simulink model "sensored_foc_model"  (R2022b)
settings: Solver=ode4  StartTime=0.0  StopTime=1800  FixedStep=50e-6  RelTol=1e-3  EnableMultiTasking=on
undefined symbols (not defined in the file or in its folder): DiscIntNeverNeededParam
libraries: slpidlib x2, spsCurrentMeasurementLib x2, mcbcontrolslib x1, spsDCVoltageSourceLib x1, eePwmGeneratorTwoLevel x1, spsPermanentMagnetSynchronousMachineLib x1, simulink x1, spsUniversalBridgeLib x1, sps_lib x1
settings Model: Creator=ASUS  LastModifiedBy=ASUS
settings SolverCC: PositivePriorityOrder=on
settings OptimizationCC: DefaultParameterBehavior=Inlined  EnhancedBackFolding=on  PassReuseOutputArgsAs=Individual arguments  ZeroExternalMemoryAtStartup=off  ZeroInternalMemoryAtStartup=off  MaxStackSize=64  OptimizeBlockOrder=speed  DifferentSizesBufferReuse=on  OptimizationCustomize=off  EfficientTunableParamExpr=on
settings DebuggingCC: ParameterTunabilityLossMsg=error
settings HardwareCC: ProdBitPerPointer=32  ProdBitPerSizeT=32  ProdBitPerPtrDiffT=32  ProdLargestAtomicFloat=None  ProdWordSize=32  ProdHWDeviceType=Custom Processor->Custom  HardwareBoardFeatureSet=SoCBlockset
settings ModelReferenceCC: ModelReferenceNumInstancesAllowed=Single
settings SFSimCC: MATLABDynamicMemAlloc=off
settings RTWCC: Description=Embedded Coder  SystemTargetFile=ert.tlc  TemplateMakefile=ert_default_tmf  GenerateReport=on  LaunchReport=on
settings CodeAppCC: ForceParamTrailComments=on  IgnoreCustomStorageClasses=off  OperatorAnnotations=on  SimulinkDataObjDesc=on  SFDataObjDesc=on  InsertBlockDesc=on
settings ERTTargetCC: InlinedParameterPlacement=NonHierarchical  ERTCustomFileTemplate=example_file_process.tlc

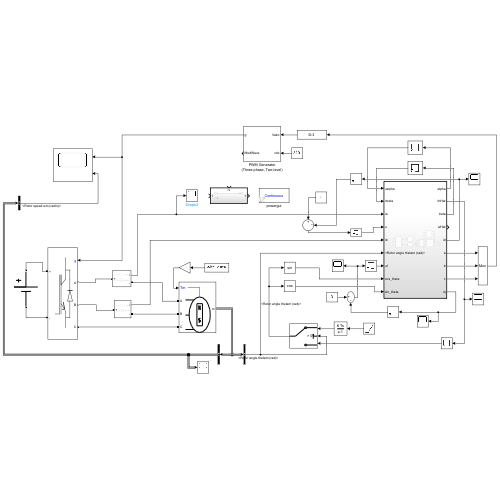
[thumbnail: Simulink's stored preview of the top-level diagram]
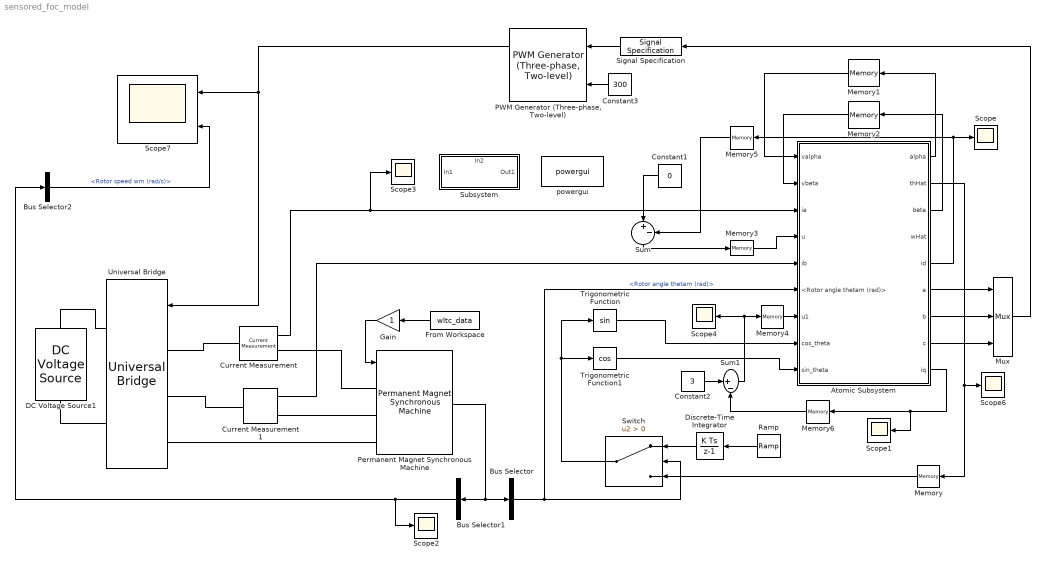
== system sensored_foc_model ==
  Atomic Subsystem : Subsystem  TreatAsAtomicUnit=on
  Bus Selector : BusSelector  OutputSignals=Rotor angle thetam (rad)  OutputAsBus=on
  Bus Selector1 : BusSelector  OutputSignals=Rotor angle thetam (rad),Rotor speed wm (rad/s),Electromagnetic torque Te (N*m)  OutputAsBus=on
  Bus Selector2 : BusSelector  OutputSignals=Rotor speed wm (rad/s)
  Constant1 : Constant  Value=0
  Constant2 : Constant  Value=3
  Constant3 : Constant  Value=300
  Current Measurement : spsCurrentMeasurementLib/Current Measurement  PhasorSimulation=off  OutputType=Complex  PSBequivalent=0
  Current Measurement1 : spsCurrentMeasurementLib/Current Measurement  PhasorSimulation=off  OutputType=Complex  PSBequivalent=0
  DC Voltage Source1 : spsDCVoltageSourceLib/DC Voltage Source  Amplitude=400  Measurements=None
  Discrete-Time Integrator : DiscreteIntegrator  SampleTime=-1  ICPrevOutput=DiscIntNeverNeededParam  ICPrevScaledInput=DiscIntNeverNeededParam
  From Workspace : FromWorkspace  VariableName=wltc_data
  Gain : Gain
  Memory{,1..6} (7 alike) : Memory
  Mux : Mux  Inputs=3
  "PWM Generator (Three-phase, Two-level)" : eePwmGeneratorTwoLevel/PWM Generator (Three-phase, Two-level)  PWMMode=Continuous PWM (CPWM)  CPWMMode=SPWM: sinusoidal PWM  DPWMMode=60 DPWM: 60 degree discontinuous PWM  fsw=1e3  Ts=5e-5
      settings: LibrarySourceBlock=|
      | ee_sl_lib/Pulse Width
      | Modulation/PWM Generator
      | (Three-phase, Two-level)
  Permanent Magnet Synchronous Machine : spsPermanentMagnetSynchronousMachineLib/Permanent Magnet Synchronous Machine  NbPhases=3  FluxDistribution=Sinusoidal  RotorType=Round  MechanicalLoad=Torque Tm  PresetModel=No  ShowDetailedParameters=on  MeasurementBus=off  Resistance=0.0485  Inductance=8.5e-3  dqInductances=[8.5e-3,8.5e-3]  La=0.000395  MachineConstant=Flux linkage established by magnets (V.s)  Flux=0.1194  VoltageCst=86.6271  TorqueCst=0.7164  Flat=120  Mechanical=[0.0027 0.0004924 4 0]  PolePairs=4  InitialConditions=[0,0, 0,0]  InitialConditions5ph=[0 0 0 0 0 0]  RefAngle=90 degrees behind phase A axis (modified Park)  IterativeDiscreteModel=Trapezoidal non iterative  TsBlock=-1  TsPowergui=0
  Ramp : simulink/Sources/Ramp  slope=0.2  start=0  InitialOutput=0
  Scope{,1..4,6} (6 alike) : Scope
  Scope7 : Scope  NumInputPorts=2
  Signal Specification : SignalSpecification  Dimensions=3
  Subsystem : Subsystem  TreatAsAtomicUnit=on
      settings: PortSchema="{\"entries\":[{\"content\":{\"sides\":[{\"content\":{\"connectorIds\":[\"In1\"]},\"type\":\"ConnectorPlacement.EquallySpacedRectSide\",\"uuid\":\"b96b767d-adbf-48c0-96dd-5b9b5a7e8c99\"},{\"content\":{\"connectorIds\":[\"Out1\"],\"side\":\"RIGHT\"},\"type\":\"ConnectorPlacement.EquallySpacedRectSide\",\"uuid\":\"f8319ca3-800b-423a-9674-6b1ed0ebf810\"},{\"content\":{\"connectorIds\":[\"In2\"],\"side\":\"TOP\"},\"type\":\"ConnectorPlacement.EquallySpacedRectSide\",\"uuid\":\"813efe85-bf04-45d5-92e6-bee0d44ebe10\"}]},\"type\":\"ConnectorPlacement.EquallySpacedConnector\",\"uuid\":\"16ba6ebc-7a04-4ed7-9949-8c258e0a29ab\"}],\"packageUris\":[\"http://schema.mathworks.com/mf0/Connector/R2020b\"],\"version\":\"1.0\"}"
      settings: LibrarySourceBlock=|
      | hdlsllib/Ports &
      | Subsystems/Subsystem
  Sum : Sum  Inputs=|+-
  Sum1 : Sum  Inputs=|+-
  Switch : Switch  Criteria=u2 > Threshold  SaturateOnIntegerOverflow=off  InputSameDT=off
  Trigonometric Function : Trigonometry
  Trigonometric Function1 : Trigonometry  Operator=cos
  Universal Bridge : spsUniversalBridgeLib/Universal Bridge  Arms=3  SnubberResistance=1e5  SnubberCapacitance=0  Device=IGBT / Diodes  Ron=1e-3  Lon=0  ForwardVoltages="[  0  0  ]"  ForwardVoltage=0  GTOparameters=[ 10e-6 , 20e-6 ]  IGBTparameters=[ 1e-6 , 2e-6 ]  Measurements=None  Measurements_2=None  converterType=Rectifier
  powergui : sps_lib/powergui  Priority=1  SimulationMode=Continuous  SampleTime=50e-6  frequency=60  Iterations=50  frequencyindice=0  Pbase=100e6  ErrMax=1e-4  UnitsV=kV  UnitsW=MW  buscounter=0  FunctionMessages=off  echomessages=off  EnableUseOfTLC=off  CurrentSourceSwitches=off  DisableSnubberDevices=off  DisableRonSwitches=off  DisableVfSwitches=off  DisplayEquations=off  AutomaticDiscreteSolvers=off  SolverType=Tustin/Backward Euler (TBE)  Interpol=off  ExternalGateDelay=off  methode=off  Ts=100  x0status=blocks  SPID=on  SwTol=0  HookPort=off  NonlinearTolerance=1e-4  nMaxIteration=100  ContinueOnMaxIteration=off  RestoreLinks=warning  ResistiveCurrentMeasurement=off  Frange=[0:2:500]  Ylog=off  Xlog=on  ShowGrid=off  save=off  variable=ZData  structure=0  ZoomFFT=off  StartTime=0.0  cycles=1  DisplayStyle=1  fundamental=60  FreqAxis=off  MaxFrequency=1000  frequencyindicesteady=1  RmsSteady=1  display=off
  wires:
  Atomic Subsystem/6(a) -> Mux/1
  "PWM Generator (Three-phase, Two-level)"/1 -> Scope7/1, Universal Bridge/1
  Signal Specification/1 -> "PWM Generator (Three-phase, Two-level)"/1
  Atomic Subsystem/3(beta) -> Memory2/1
  Mux/1 -> Signal Specification/1
  Current Measurement1/1 -> Atomic Subsystem/5(ib)
  Constant3/1 -> "PWM Generator (Three-phase, Two-level)"/2
  Atomic Subsystem/7(b) -> Mux/2
  Bus Selector/1 -> Switch/2, Atomic Subsystem/6(<Rotor angle thetam (rad)>)  "<Rotor angle thetam (rad)>"
  Trigonometric Function1/1 -> Atomic Subsystem/9(sin_theta)
  Current Measurement/1 -> Scope3/1, Atomic Subsystem/3(ia)
  Ramp/1 -> Discrete-Time Integrator/1
  Atomic Subsystem/8(c) -> Mux/3
  Memory1/1 -> Atomic Subsystem/1(valpha)
  Permanent Magnet Synchronous Machine/1 -> Bus Selector1/1, Bus Selector/1
  Discrete-Time Integrator/1 -> Switch/1
  Switch/1 -> Trigonometric Function/1, Trigonometric Function1/1
  Constant1/1 -> Sum/1
  Memory2/1 -> Atomic Subsystem/2(vbeta)
  Memory/1 -> Switch/3
  Atomic Subsystem/1(alpha) -> Memory1/1
  Atomic Subsystem/9(iq) -> Scope1/1, Memory6/1
  Trigonometric Function/1 -> Atomic Subsystem/8(cos_theta)
  Constant2/1 -> Sum1/1
  Atomic Subsystem/2(thHat) -> Memory/1, Scope6/1
  Atomic Subsystem/5(id) -> Scope/1, Memory5/1
  Memory3/1 -> Atomic Subsystem/4(u)
  Sum/1 -> Memory3/1
  Memory4/1 -> Atomic Subsystem/7(u1)
  Sum1/1 -> Memory4/1, Scope4/1
  Memory5/1 -> Sum/2
  Memory6/1 -> Sum1/2
  Bus Selector1/1 -> Bus Selector2/1, Scope2/1
  Bus Selector2/1 -> Scope7/2  "<Rotor speed wm (rad/s)>"
  From Workspace/1 -> Gain/1
  Gain/1 -> Permanent Magnet Synchronous Machine/1
  connections:
  DC Voltage Source1/LConn1 -- Universal Bridge/RConn2
  DC Voltage Source1/RConn1 -- Universal Bridge/RConn1
  Universal Bridge/LConn1 -- Current Measurement/LConn1
  Universal Bridge/LConn2 -- Current Measurement1/LConn1
  Universal Bridge/LConn3 -- Permanent Magnet Synchronous Machine/LConn3
  Current Measurement/RConn1 -- Permanent Magnet Synchronous Machine/LConn1
  Current Measurement1/RConn1 -- Permanent Magnet Synchronous Machine/LConn2

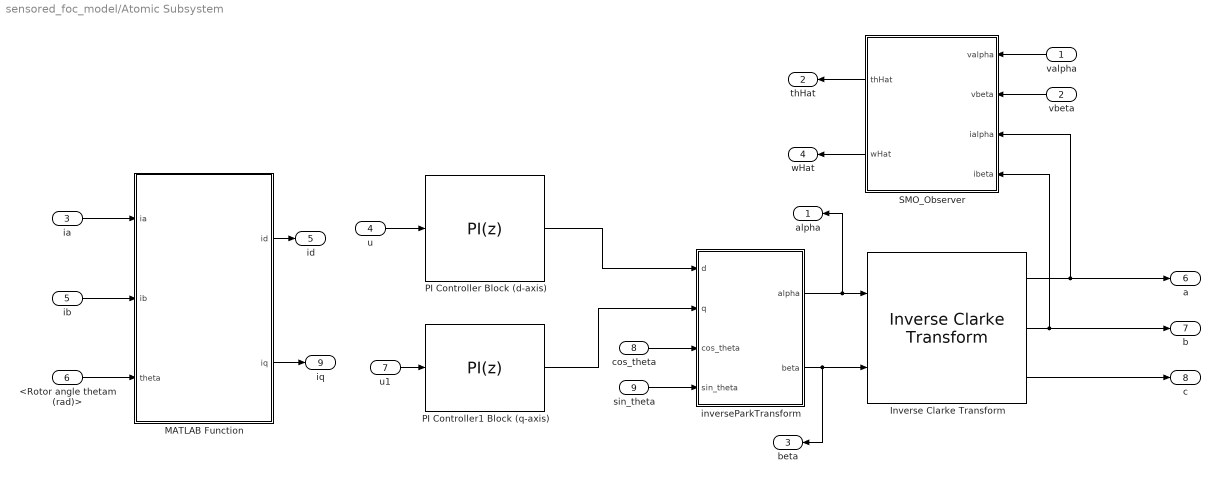
== system sensored_foc_model/Atomic Subsystem ==
  valpha : Inport
  vbeta : Inport  Port=2
  ia : Inport  Port=3
  u : Inport  Port=4
  ib : Inport  Port=5
  <Rotor angle thetam (rad)> : Inport  Port=6
  u1 : Inport  Port=7
  cos_theta : Inport  Port=8
  sin_theta : Inport  Port=9
  Inverse Clarke Transform : mcbcontrolslib/Inverse Clarke Transform
      settings: LibrarySourceBlock=mcbhdllib/Controls/Math Transforms/Inverse Clarke Transform
  MATLAB Function : MATLAB Function  TreatAsAtomicUnit=on
  PI Controller Block (d-axis) : slpidlib/PID Controller  Controller=PI  Form=Parallel  TimeDomain=Discrete-time  UseExternalTs=off  SampleTime=50e-6  IntegratorMethod=Forward Euler  FilterMethod=Forward Euler  ControllerParametersSource=internal  P=4.5  I=400  UseKiTs=on  D=0  N=100  UseFilter=on  TunerSelectOption=Transfer Function Based (PID Tuner App)  InitialConditionSource=internal  InitialConditionForIntegrator=0  InitialConditionForFilter=0  DifferentiatorICPrevScaledInput=0  ExternalReset=none  TrackingMode=off  Kt=1  LimitOutput=on  SatLimitsSource=internal  UpperSaturationLimit=300  LowerSaturationLimit=-300  LinearizeAsGain=on  AntiWindupMode=clamping  Kb=1  LimitIntegrator=off  UpperIntegratorSaturationLimit=inf  LowerIntegratorSaturationLimit=-inf  RndMeth=Simplest  POutMin=10  POutMax=20  IOutMin=100  IOutMax=500  DOutMin=[]  DOutMax=[]  NOutMin=[]  NOutMax=[]  SumOutMin=[]  SumOutMax=[]  SaturationOutDataTypeStr=Inherit: Inherit via back propagation  SaturationOutMin=[]  SaturationOutMax=[]  PParamMin=[]  PParamMax=[]  IParamMin=[]  IParamMax=[]  DParamMin=[]  DParamMax=[]  NParamMin=[]  NParamMax=[]  KbParamMin=[]  KbParamMax=[]  KtParamMin=[]  KtParamMax=[]  KbOutMin=[]  KbOutMax=[]  KtOutMin=[]  KtOutMax=[]  IntegratorOutMin=[]  IntegratorOutMax=[]  FilterOutMin=[]  FilterOutMax=[]  SumI1OutMin=[]  SumI1OutMax=[]  SumI2OutMin=[]  SumI2OutMax=[]  SumI3OutMin=[]  SumI3OutMax=[]  SumI4OutMin=[]  SumI4OutMax=[]  SumDOutMin=[]  SumDOutMax=[]  DifferentiatorOutMin=[]  DifferentiatorOutMax=[]  FilterDiffOutCoefMin=[]  FilterDiffOutCoefMax=[]  ReciprocalOutMin=[]  ReciprocalOutMax=[]  SumDenOutMin=[]  SumDenOutMax=[]  SumNumOutMin=[]  SumNumOutMax=[]  DivideOutMin=[]  DivideOutMax=[]  UdiffTsProdOutMin=[]  UdiffTsProdOutMax=[]  NTsProdOutMin=[]  NTsProdOutMax=[]  UintegralTsProdOutMin=[]  UintegralTsProdOutMax=[]  UngainTsProdOutMin=[]  UngainTsProdOutMax=[]  ClampingZeroOutDataTypeStr=Inherit: Inherit via back propagation  ClampingZeroOutMin=[]  ClampingZeroOutMax=[]  FilterDenConstantOutDataTypeStr=Inherit: Inherit via back propagation  FilterDenConstantOutMin=[]  FilterDenConstantOutMax=[]  PCopyOutDataTypeStr=Inherit: Inherit via back propagation  PCopyOutMin=[]  PCopyOutMax=[]  NCopyOutDataTypeStr=Inherit: Inherit via back propagation  NCopyOutMin=[]  NCopyOutMax=[]  IntegratorContinuousStateAttributes=''  IntegratorStateMustResolveToSignalObject=off  IntegratorRTWStateStorageClass=Auto  FilterContinuousStateAttributes=''  FilterStateMustResolveToSignalObject=off  FilterRTWStateStorageClass=Auto  ParallelPVariant=InternalParameters  IdealPVariant=Disabled  IVariant=InternalParameters  DVariant=Disabled  IntegratorVariant=Discrete  SatVariant=Enabled  AWVariant=DiscClampingParallel  PCopyVariant=Disabled  TRVariant=Disabled  FdbkBlocksVariant=Forward  IdealPFdbkVariant=Disabled  SatFdbkVariant=Disabled  DerivativeFilterVariant=Disabled  NVariant=Disabled  NCopyVariant=Disabled_SignalSpec  FilterICVariant=Disabled  IntegratorICVariant=InternalICs  ExternalResetVariant=Disabled  TRSumVariant=Passthrough  SumFdbkVariant=Disabled  SumVariant=Sum_PI  TsampFilterVariant=InternalTs  TsampNgainVariant=Passthrough  TsampIntegralVariant=Passthrough  ExternalSaturationOutDataTypeStr=Inherit: Same as second input
      settings: LibrarySourceBlock=mcbhdllib/Controls/Controllers/PI Controller
  PI Controller1 Block (q-axis) : slpidlib/PID Controller  Controller=PI  Form=Parallel  TimeDomain=Discrete-time  UseExternalTs=off  SampleTime=50e-6  IntegratorMethod=Forward Euler  FilterMethod=Forward Euler  ControllerParametersSource=internal  P=4.5  I=400  UseKiTs=on  D=0  N=100  UseFilter=on  TunerSelectOption=Transfer Function Based (PID Tuner App)  InitialConditionSource=internal  InitialConditionForIntegrator=0  InitialConditionForFilter=0  DifferentiatorICPrevScaledInput=0  ExternalReset=none  TrackingMode=off  Kt=1  LimitOutput=on  SatLimitsSource=internal  UpperSaturationLimit=300  LowerSaturationLimit=-300  LinearizeAsGain=on  AntiWindupMode=clamping  Kb=1  LimitIntegrator=off  UpperIntegratorSaturationLimit=inf  LowerIntegratorSaturationLimit=-inf  RndMeth=Simplest  POutMin=10  POutMax=20  IOutMin=100  IOutMax=500  DOutMin=[]  DOutMax=[]  NOutMin=[]  NOutMax=[]  SumOutMin=[]  SumOutMax=[]  SaturationOutDataTypeStr=Inherit: Inherit via back propagation  SaturationOutMin=[]  SaturationOutMax=[]  PParamMin=[]  PParamMax=[]  IParamMin=[]  IParamMax=[]  DParamMin=[]  DParamMax=[]  NParamMin=[]  NParamMax=[]  KbParamMin=[]  KbParamMax=[]  KtParamMin=[]  KtParamMax=[]  KbOutMin=[]  KbOutMax=[]  KtOutMin=[]  KtOutMax=[]  IntegratorOutMin=[]  IntegratorOutMax=[]  FilterOutMin=[]  FilterOutMax=[]  SumI1OutMin=[]  SumI1OutMax=[]  SumI2OutMin=[]  SumI2OutMax=[]  SumI3OutMin=[]  SumI3OutMax=[]  SumI4OutMin=[]  SumI4OutMax=[]  SumDOutMin=[]  SumDOutMax=[]  DifferentiatorOutMin=[]  DifferentiatorOutMax=[]  FilterDiffOutCoefMin=[]  FilterDiffOutCoefMax=[]  ReciprocalOutMin=[]  ReciprocalOutMax=[]  SumDenOutMin=[]  SumDenOutMax=[]  SumNumOutMin=[]  SumNumOutMax=[]  DivideOutMin=[]  DivideOutMax=[]  UdiffTsProdOutMin=[]  UdiffTsProdOutMax=[]  NTsProdOutMin=[]  NTsProdOutMax=[]  UintegralTsProdOutMin=[]  UintegralTsProdOutMax=[]  UngainTsProdOutMin=[]  UngainTsProdOutMax=[]  ClampingZeroOutDataTypeStr=Inherit: Inherit via back propagation  ClampingZeroOutMin=[]  ClampingZeroOutMax=[]  FilterDenConstantOutDataTypeStr=Inherit: Inherit via back propagation  FilterDenConstantOutMin=[]  FilterDenConstantOutMax=[]  PCopyOutDataTypeStr=Inherit: Inherit via back propagation  PCopyOutMin=[]  PCopyOutMax=[]  NCopyOutDataTypeStr=Inherit: Inherit via back propagation  NCopyOutMin=[]  NCopyOutMax=[]  IntegratorContinuousStateAttributes=''  IntegratorStateMustResolveToSignalObject=off  IntegratorRTWStateStorageClass=Auto  FilterContinuousStateAttributes=''  FilterStateMustResolveToSignalObject=off  FilterRTWStateStorageClass=Auto  ParallelPVariant=InternalParameters  IdealPVariant=Disabled  IVariant=InternalParameters  DVariant=Disabled  IntegratorVariant=Discrete  SatVariant=Enabled  AWVariant=DiscClampingParallel  PCopyVariant=Disabled  TRVariant=Disabled  FdbkBlocksVariant=Forward  IdealPFdbkVariant=Disabled  SatFdbkVariant=Disabled  DerivativeFilterVariant=Disabled  NVariant=Disabled  NCopyVariant=Disabled_SignalSpec  FilterICVariant=Disabled  IntegratorICVariant=InternalICs  ExternalResetVariant=Disabled  TRSumVariant=Passthrough  SumFdbkVariant=Disabled  SumVariant=Sum_PI  TsampFilterVariant=InternalTs  TsampNgainVariant=Passthrough  TsampIntegralVariant=Passthrough  ExternalSaturationOutDataTypeStr=Inherit: Same as second input
      settings: LibrarySourceBlock=mcbhdllib/Controls/Controllers/PI Controller
  SMO_Observer : MATLAB Function  TreatAsAtomicUnit=on
  inverseParkTransform : MATLAB Function  TreatAsAtomicUnit=on
  alpha : Outport
  thHat : Outport  Port=2
  beta : Outport  Port=3
  wHat : Outport  Port=4
  id : Outport  Port=5
  a : Outport  Port=6
  b : Outport  Port=7
  c : Outport  Port=8
  iq : Outport  Port=9
  wires:
  cos_theta/1 -> inverseParkTransform/3(cos_theta)
  PI Controller1 Block (q-axis)/1 -> inverseParkTransform/2(q)
  Inverse Clarke Transform/2 -> b/1, SMO_Observer/4(ibeta)
  Inverse Clarke Transform/1 -> a/1, SMO_Observer/3(ialpha)
  ia/1 -> MATLAB Function/1(ia)
  SMO_Observer/2(wHat) -> wHat/1
  inverseParkTransform/1(alpha) -> alpha/1, Inverse Clarke Transform/1
  inverseParkTransform/2(beta) -> beta/1, Inverse Clarke Transform/2
  PI Controller Block (d-axis)/1 -> inverseParkTransform/1(d)
  MATLAB Function/2(iq) -> iq/1
  MATLAB Function/1(id) -> id/1
  Inverse Clarke Transform/3 -> c/1
  u/1 -> PI Controller Block (d-axis)/1
  u1/1 -> PI Controller1 Block (q-axis)/1
  SMO_Observer/1(thHat) -> thHat/1
  valpha/1 -> SMO_Observer/1(valpha)
  ib/1 -> MATLAB Function/2(ib)
  vbeta/1 -> SMO_Observer/2(vbeta)
  <Rotor angle thetam (rad)>/1 -> MATLAB Function/3(theta)
  sin_theta/1 -> inverseParkTransform/4(sin_theta)

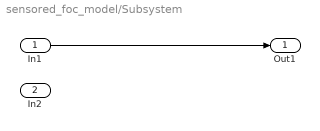
== system sensored_foc_model/Subsystem ==
  In1 : Inport
  In2 : Inport  Port=2
  Out1 : Outport
  wires:
  In1/1 -> Out1/1

== matlab function sensored_foc_model/Atomic Subsystem/SMO_Observer ==
  settings: updateMethod=DISCRETE  sampleTime=1/20e3
  data: valpha input; thHat output; vbeta input; ialpha input; ibeta input; wHat output
function [thHat, wHat] = smo(valpha, vbeta, ialpha, ibeta)
    %#codegen
    persistent ia_est ib_est z_alpha z_beta th_est w_est
    
    if isempty(ia_est)
        ia_est = 0; ib_est = 0; 
        z_alpha = 0; z_beta = 0;
        th_est = 0; w_est = 62.8; 
    end
    
    % Exact plant parameters from the machine block mask
    Rs = 0.0485; Ls = 0.000395; Ts = 1 / 20e3;
    p = 4;          % 4 pole pairs
    k = 30.0;       % Stable sliding gain
    wc = 2000;      % Stable filter cutoff frequency
    
    % Current estimation dynamics in stationary alpha-beta frame
    ia_est = ia_est + (Ts / Ls) * (valpha - Rs * ia_est - z_alpha);
    ib_est = ib_est + (Ts / Ls) * (vbeta - Rs * ib_est - z_beta);
    
    % Sliding surfaces with boundary layer chattering mitigation
    s_alpha = ia_est - ialpha;
    s_beta  = ib_est - ibeta;
    
    eps_bl = 0.05;
    v_alpha_sw = k * (s_alpha / (abs(s_alpha) + eps_bl));
    v_beta_sw  = k * (s_beta  / (abs(s_beta) + eps_bl));
    
    % Low-pass filtered back-EMF extraction
    z_alpha = z_alpha + Ts * wc * (v_alpha_sw - z_alpha);
    z_beta  = z_beta  + Ts * wc * (v_beta_sw  - z_beta);
    
    % Raw electrical angle extraction
    th_raw = atan2(-z_alpha, z_beta);
    
    % Software PLL phase error tracking
    th_err = atan2(sin(th_raw - th_est), cos(th_raw - th_est));
    
    kp_pll = 100;
    ki_pll = 2000;
    
    w_est = w_est + Ts * ki_pll * th_err;
    w_est = max(min(w_est, 1000), -1000); 
    
    th_est = th_est + Ts * (w_est + kp_pll * th_err);
    
    % Final normalized output angle and speed estimation
    thHat = atan2(sin(th_est), cos(th_est));
    wHat = w_est;
end

== matlab function sensored_foc_model/Atomic Subsystem/MATLAB Function ==
  data: ia input; id output; ib input; theta input; iq output
function [id, iq] = transforms(ia, ib, theta)
    %#codegen
    ialpha = ia;
    ibeta = (ia + 2 * ib) / sqrt(3);
    c = cos(theta);
    s = sin(theta);
    id = ialpha * c + ibeta * s;
    iq = -ialpha * s + ibeta * c;
end

== matlab function sensored_foc_model/Atomic Subsystem/inverseParkTransform ==
  data: d input; alpha output; q input; cos_theta input; sin_theta input; beta output
function [alpha, beta] = fcn(d, q, cos_theta, sin_theta)
%#codegen
alpha = d * cos_theta - q * sin_theta;
beta  = d * sin_theta + q * cos_theta;
end
